simulink model "LinearizedModel"  (R2026b)
settings: Solver=VariableStepAuto
undefined symbols (not defined in the file): As, Bs, Cs, Ds, nom
settings Model: Creator=Mauro  LastModifiedBy=Mauro

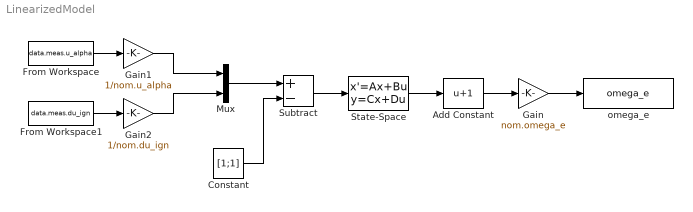
== system LinearizedModel ==
  Add Constant : Bias  Bias=1  SaturateOnIntegerOverflow=off
  Constant : Constant  Value=[1;1]
  From Workspace : FromWorkspace  VariableName=data.meas.u_alpha
  From Workspace1 : FromWorkspace  VariableName=data.meas.du_ign
  Gain : Gain  Gain=nom.omega_e
  Gain1 : Gain  Gain=1/nom.u_alpha
  Gain2 : Gain  Gain=1/nom.du_ign
  Mux : Mux  Inputs=2
  State-Space : StateSpace  A=As  B=Bs  C=Cs  D=Ds  InitialCondition=0
  Subtract : Sum  Inputs=+-
  omega_e : ToWorkspace  VariableName=omega_e  SaveFormat=Timeseries  SampleTime=-1
  wires:
  Subtract/1 -> State-Space/1
  Constant/1 -> Subtract/2
  State-Space/1 -> Add Constant/1
  Add Constant/1 -> Gain/1
  Gain/1 -> omega_e/1
  Mux/1 -> Subtract/1
  From Workspace/1 -> Gain1/1
  From Workspace1/1 -> Gain2/1
  Gain2/1 -> Mux/2
  Gain1/1 -> Mux/1
